simulink model "Lab1_3_1_2_Feedforward"  (R2024b)
settings: Solver=ode5  StartTime=0.0  StopTime=3  FixedStep=1e-03  RelTol=1e-3
undefined symbols (not defined in the file): BEMF_comp, delta_i, drv, gbox, Inertia_comp, Kd, Ki, Kp, Kw, mot, N2Beq, National_Instruments, PCI, sens, Tau_sf, TL, wc, wc2
libraries: sldrtlib x2
settings Model: SimulationMode=external  ExtModeTrigDuration=45001  Creator=lenovo  LastModifiedBy=aboulenien
settings DataIOCC: ReturnWorkspaceOutputs=off
settings HardwareCC: ProdBitPerLong=64  ProdHWDeviceType=Intel->x86-64 (Linux 64)
settings RTWCC: Description=Simulink Desktop Real-Time  SystemTargetFile=sldrt.tlc  TemplateMakefile=sldrt.tmf  RTWCompilerOptimization=on
settings CodeAppCC: MaxIdLength=95
settings SimulinkDesktopRealTimeCC: TargetLibSuffix=_sldrt.a  TargetPreCompLibLocation=C:\Program Files\MATLAB\R2024b\toolbox\sldrt\lib\win64  ParMdlRefBuildCompliant=on

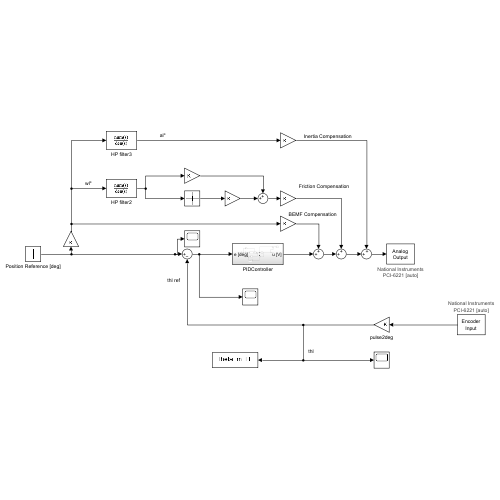
[thumbnail: Simulink's stored preview of the top-level diagram]
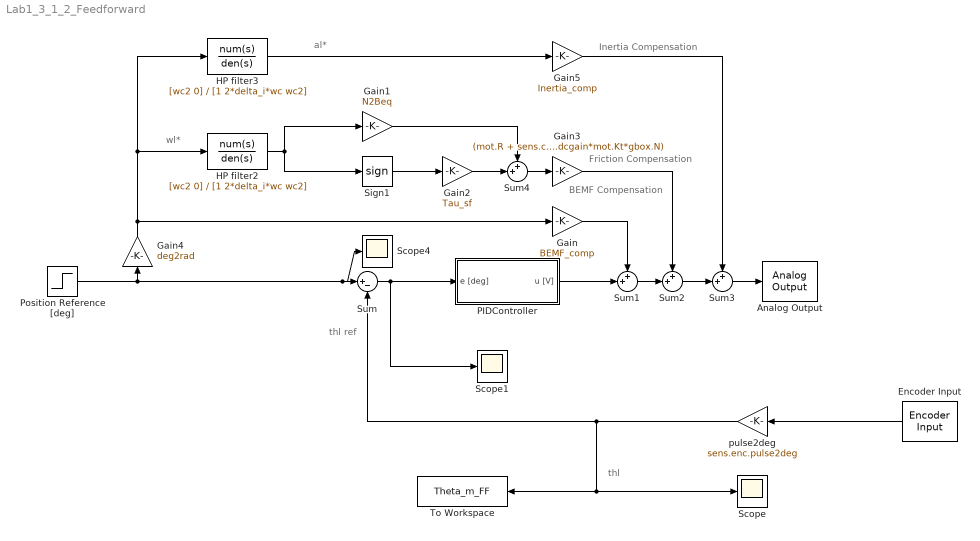
== system Lab1_3_1_2_Feedforward ==
  note: Inertia Compensation
  note: al*
  note: BEMF Compensation
  note: Friction Compensation
  note: thl
  note: thl ref
  note: wl*
  Analog Output : sldrtlib/Analog Output  SampleTime=-1  MaxMissedTicks=10  ShowMissedTicks=off  YieldWhenWaiting=off  DrvName=National_Instruments/PCI-6221  DrvAddress=4294967295  DrvOptions=[0 0 0 2 0]  Channels=1  RangeMode=1  VoltRange=1  InitialValue=0  FinalValue=0
      settings: AttributesFormatString=National Instruments\nPCI-6221 [auto]
  Encoder Input : sldrtlib/Encoder Input  SampleTime=-1  MaxMissedTicks=10  ShowMissedTicks=off  YieldWhenWaiting=off  DrvName=National_Instruments/PCI-6221  DrvAddress=4294967295  DrvOptions=[0 0 0 2 0]  Channels=1  QuadMode=3  IndexPulse=1  InputFilter=Inf  DataType=1
      settings: AttributesFormatString=National Instruments\nPCI-6221 [auto]
  Gain : Gain  Gain=BEMF_comp
  Gain1 : Gain  Gain=N2Beq
  Gain2 : Gain  Gain=Tau_sf
  Gain3 : Gain  Gain=(mot.R + sens.curr.Rs)/(drv.dcgain*mot.Kt*gbox.N)
  Gain4 : Gain  Gain=deg2rad
  Gain5 : Gain  Gain=Inertia_comp
  HP filter2 : TransferFcn  Numerator=[wc2 0]  Denominator=[1 2*delta_i*wc wc2]
  HP filter3 : TransferFcn  Numerator=[wc2 0]  Denominator=[1 2*delta_i*wc wc2]
  PIDController : Subsystem
  Position Reference [deg] : Step  After=360  SampleTime=0
  Scope : Scope
  Scope1 : Scope
  Scope4 : Scope
  Sign1 : Signum
  Sum : Sum  Inputs=|+-
  Sum{1..4} (4 alike) : Sum  Inputs=++|
  To Workspace : ToWorkspace  VariableName=Theta_m_FF  SaveFormat=Structure With Time  SampleTime=0.001
  pulse2deg : Gain  Gain=sens.enc.pulse2deg
  wires:
  Sum3/1 -> Analog Output/1
  Encoder Input/1 -> pulse2deg/1
  Gain2/1 -> Sum4/2
  Sum4/1 -> Gain3/1
  Gain1/1 -> Sum4/1
  Gain3/1 -> Sum2/1
  Sign1/1 -> Gain2/1
  Gain5/1 -> Sum3/1
  Sum1/1 -> Sum2/2
  pulse2deg/1 -> Scope/1, To Workspace/1, Sum/2
  Gain/1 -> Sum1/1
  Sum2/1 -> Sum3/2
  PIDController/1(u [V]) -> Sum1/2
  Sum/1 -> PIDController/1(e [deg]), Scope1/1
  Gain4/1 -> HP filter3/1, HP filter2/1, Gain/1
  Position Reference [deg]/1 -> Scope4/1, Sum/1, Gain4/1
  HP filter2/1 -> Gain1/1, Sign1/1
  HP filter3/1 -> Gain5/1

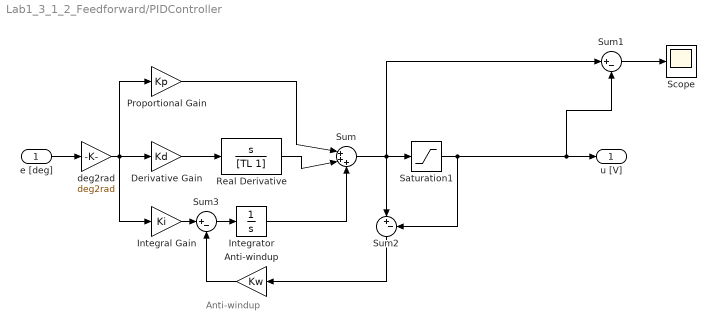
== system Lab1_3_1_2_Feedforward/PIDController ==
  note: Anti-windup
  e [deg] : Inport
  Anti-windup : Gain  Gain=Kw
  Derivative Gain : Gain  Gain=Kd
  Integral Gain : Gain  Gain=Ki
  Integrator : Integrator
  Proportional Gain : Gain  Gain=Kp
  Real Derivative : TransferFcn  Numerator=[1 0]  Denominator=[TL 1]
  Saturation1 : Saturate  UpperLimit=12  LowerLimit=-12
  Scope : Scope
  Sum : Sum  Inputs=|+++
  Sum1 : Sum  Inputs=|+-
  Sum2 : Sum  Inputs=|+-
  Sum3 : Sum  Inputs=|+-
  deg2rad : Gain  Gain=deg2rad
  u [V] : Outport
  wires:
  Saturation1/1 -> Sum2/2, Sum1/2, u [V]/1
  Sum1/1 -> Scope/1
  deg2rad/1 -> Derivative Gain/1, Integral Gain/1, Proportional Gain/1
  e [deg]/1 -> deg2rad/1
  Proportional Gain/1 -> Sum/1
  Derivative Gain/1 -> Real Derivative/1
  Real Derivative/1 -> Sum/2
  Integrator/1 -> Sum/3
  Sum2/1 -> Anti-windup/1
  Integral Gain/1 -> Sum3/1
  Sum3/1 -> Integrator/1
  Anti-windup/1 -> Sum3/2
  Sum/1 -> Sum1/1, Sum2/1, Saturation1/1
